simulink model "single_phase_ttype_inverter_param"  (R2026a)
settings: Solver=ode23tb  StopTime=param.sim.simlength  FixedStep=tc  MaxStep=param.glb_time.tc
values from neighbouring files (symbols this model uses):
  param = add_template_extras(param, options)    [init_model.m]
undefined symbols (not defined in the file or in its folder): delta_fht1, Ld_fht1, omega_fht1, ts_inv, Vac_FS, Vdc_nom, Xbez
libraries: fl_lib x36, nesl_utility x18, single_phase_transformer_lib x3, phase_shift_filter_ccaller x2, dclink_for_three_levels x1, three_phase_voltage_emulator x1, power_meter_iec x1, single_phase_transformer x1, three_phase_diode_rectifier x1, three_phase_diode_rectifier_with_thermal_model x1, full_bridge_three_level_ttype_ideal_switch_based_model x1, full_bridge_three_level_ttype_mosfet_based_model x1
(part 3 of 4)

== system single_phase_ttype_inverter_param/single_phase_inverter/single phase inverter control/single_phase_inverter_ctrl/phase generator/dq_pll_ccaller/first_harmonic_tracker1 ==
  u : Inport
  Bus Selector : BusSelector  OutputSignals=output_pu_hat
  Constant : Constant  Value=param.glb_time.ts_inv
  Constant1 : Constant  Value=0
  Constant2 : Constant  Value=param.afe.ctrl.fht_grid.omega_fht
  Constant3 : Constant  Value=param.afe.ctrl.fht_grid.delta_fht
  Constant4 : Constant  Value=param.afe.ctrl.fht_grid.Ld_fht(1)
  Constant5 : Constant  Value=param.afe.ctrl.fht_grid.Ld_fht(2)
  Data Type Conversion{1..2,6..9} (6 alike) : DataTypeConversion  OutDataTypeStr=single  SaturateOnIntegerOverflow=off  RndMeth=Floor
  Data Type Conversion3 : DataTypeConversion  OutDataTypeStr=uint8  SaturateOnIntegerOverflow=off  RndMeth=Floor
  Data Type Conversion4 : DataTypeConversion  OutDataTypeStr=double  SaturateOnIntegerOverflow=off  RndMeth=Floor
  Data Type Conversion5 : DataTypeConversion  OutDataTypeStr=uint8  SaturateOnIntegerOverflow=off  RndMeth=Floor
  Step : Step  Time=0.0125  InitialValue=1  FinalValue=0
  first_harmonic_tracker : CCaller  FunctionName=first_harmonic_tracker_process_simulink  PortSpecificationStruct="%)30     .    B \\   8    (     @         %    \"     D    !     0         %  0 \"0    $    _    07)G3F%M90  4&]R=$YA;64 4V-O<&4     26YD97@     5'EP90      4VEZ90      27-';&]B86P   X    P    !@    @    $          4    (     0    ,    !         !   P!O=70 #@   #     &    \"     0         !0    @    !     P    $         $  # &]U=  .    .     8    (    !          %    \"     $    &     0         0  ...(+4988 chars)"
  u_hat : Outport
  wires:
  Data Type Conversion4/1 -> u_hat/1
  Data Type Conversion3/1 -> first_harmonic_tracker/1
  Data Type Conversion1/1 -> first_harmonic_tracker/3
  Data Type Conversion2/1 -> first_harmonic_tracker/2
  first_harmonic_tracker/1 -> Bus Selector/1
  Bus Selector/1 -> Data Type Conversion4/1  "<output_pu_hat>"
  Step/1 -> Data Type Conversion3/1
  u/1 -> Data Type Conversion2/1
  Constant/1 -> Data Type Conversion1/1
  Constant1/1 -> Data Type Conversion5/1
  Data Type Conversion5/1 -> first_harmonic_tracker/8
  Constant2/1 -> Data Type Conversion6/1
  Data Type Conversion6/1 -> first_harmonic_tracker/4
  Constant3/1 -> Data Type Conversion7/1
  Data Type Conversion7/1 -> first_harmonic_tracker/5
  Constant4/1 -> Data Type Conversion8/1
  Data Type Conversion8/1 -> first_harmonic_tracker/6
  Constant5/1 -> Data Type Conversion9/1
  Data Type Conversion9/1 -> first_harmonic_tracker/7

== system single_phase_ttype_inverter_param/single_phase_inverter/single phase inverter control/single_phase_inverter_ctrl/phase generator/dq_pll_ccaller/first_harmonic_tracker2 ==
  u : Inport
  Bus Selector : BusSelector  OutputSignals=output_pu_hat
  Constant : Constant  Value=param.glb_time.ts_inv
  Constant1 : Constant  Value=2
  Constant2 : Constant  Value=param.afe.ctrl.fht_grid.omega_fht
  Constant3 : Constant  Value=param.afe.ctrl.fht_grid.delta_fht
  Constant4 : Constant  Value=param.afe.ctrl.fht_grid.Ld_fht(1)
  Constant5 : Constant  Value=param.afe.ctrl.fht_grid.Ld_fht(2)
  Data Type Conversion{1..2,6..9} (6 alike) : DataTypeConversion  OutDataTypeStr=single  SaturateOnIntegerOverflow=off  RndMeth=Floor
  Data Type Conversion3 : DataTypeConversion  OutDataTypeStr=uint8  SaturateOnIntegerOverflow=off  RndMeth=Floor
  Data Type Conversion4 : DataTypeConversion  OutDataTypeStr=double  SaturateOnIntegerOverflow=off  RndMeth=Floor
  Data Type Conversion5 : DataTypeConversion  OutDataTypeStr=uint8  SaturateOnIntegerOverflow=off  RndMeth=Floor
  Step : Step  Time=0.0125  InitialValue=1  FinalValue=0
  first_harmonic_tracker : CCaller  FunctionName=first_harmonic_tracker_process_simulink  PortSpecificationStruct="%)30     .    B \\   8    (     @         %    \"     D    !     0         %  0 \"0    $    _    07)G3F%M90  4&]R=$YA;64 4V-O<&4     26YD97@     5'EP90      4VEZ90      27-';&]B86P   X    P    !@    @    $          4    (     0    ,    !         !   P!O=70 #@   #     &    \"     0         !0    @    !     P    $         $  # &]U=  .    .     8    (    !          %    \"     $    &     0         0  ...(+4988 chars)"
  u_hat : Outport
  wires:
  Data Type Conversion9/1 -> first_harmonic_tracker/7
  Constant5/1 -> Data Type Conversion9/1
  Data Type Conversion8/1 -> first_harmonic_tracker/6
  Constant4/1 -> Data Type Conversion8/1
  Data Type Conversion7/1 -> first_harmonic_tracker/5
  Constant3/1 -> Data Type Conversion7/1
  Data Type Conversion6/1 -> first_harmonic_tracker/4
  Constant2/1 -> Data Type Conversion6/1
  Data Type Conversion5/1 -> first_harmonic_tracker/8
  Constant1/1 -> Data Type Conversion5/1
  Constant/1 -> Data Type Conversion1/1
  u/1 -> Data Type Conversion2/1
  Step/1 -> Data Type Conversion3/1
  Bus Selector/1 -> Data Type Conversion4/1  "<output_pu_hat>"
  first_harmonic_tracker/1 -> Bus Selector/1
  Data Type Conversion2/1 -> first_harmonic_tracker/2
  Data Type Conversion1/1 -> first_harmonic_tracker/3
  Data Type Conversion3/1 -> first_harmonic_tracker/1
  Data Type Conversion4/1 -> u_hat/1

== system single_phase_ttype_inverter_param/single_phase_inverter/single phase inverter control/single_phase_inverter_ctrl/phase generator/dq_pll_ccaller/first_harmonic_tracker3 ==
  u : Inport
  Bus Selector : BusSelector  OutputSignals=output_pu_hat
  Constant : Constant  Value=param.glb_time.ts_inv
  Constant1 : Constant  Value=4
  Constant2 : Constant  Value=param.afe.ctrl.fht_grid.omega_fht
  Constant3 : Constant  Value=param.afe.ctrl.fht_grid.delta_fht
  Constant4 : Constant  Value=param.afe.ctrl.fht_grid.Ld_fht(1)
  Constant5 : Constant  Value=param.afe.ctrl.fht_grid.Ld_fht(2)
  Data Type Conversion{1..2,6..9} (6 alike) : DataTypeConversion  OutDataTypeStr=single  SaturateOnIntegerOverflow=off  RndMeth=Floor
  Data Type Conversion3 : DataTypeConversion  OutDataTypeStr=uint8  SaturateOnIntegerOverflow=off  RndMeth=Floor
  Data Type Conversion4 : DataTypeConversion  OutDataTypeStr=double  SaturateOnIntegerOverflow=off  RndMeth=Floor
  Data Type Conversion5 : DataTypeConversion  OutDataTypeStr=uint8  SaturateOnIntegerOverflow=off  RndMeth=Floor
  Step : Step  Time=0.0125  InitialValue=1  FinalValue=0
  first_harmonic_tracker : CCaller  FunctionName=first_harmonic_tracker_process_simulink  PortSpecificationStruct="%)30     .    B \\   8    (     @         %    \"     D    !     0         %  0 \"0    $    _    07)G3F%M90  4&]R=$YA;64 4V-O<&4     26YD97@     5'EP90      4VEZ90      27-';&]B86P   X    P    !@    @    $          4    (     0    ,    !         !   P!O=70 #@   #     &    \"     0         !0    @    !     P    $         $  # &]U=  .    .     8    (    !          %    \"     $    &     0         0  ...(+4988 chars)"
  u_hat : Outport
  wires:
  Data Type Conversion4/1 -> u_hat/1
  Data Type Conversion3/1 -> first_harmonic_tracker/1
  Data Type Conversion1/1 -> first_harmonic_tracker/3
  Data Type Conversion2/1 -> first_harmonic_tracker/2
  first_harmonic_tracker/1 -> Bus Selector/1
  Bus Selector/1 -> Data Type Conversion4/1  "<output_pu_hat>"
  Step/1 -> Data Type Conversion3/1
  u/1 -> Data Type Conversion2/1
  Constant/1 -> Data Type Conversion1/1
  Constant1/1 -> Data Type Conversion5/1
  Data Type Conversion5/1 -> first_harmonic_tracker/8
  Constant2/1 -> Data Type Conversion6/1
  Data Type Conversion6/1 -> first_harmonic_tracker/4
  Constant3/1 -> Data Type Conversion7/1
  Data Type Conversion7/1 -> first_harmonic_tracker/5
  Constant4/1 -> Data Type Conversion8/1
  Data Type Conversion8/1 -> first_harmonic_tracker/6
  Constant5/1 -> Data Type Conversion9/1
  Data Type Conversion9/1 -> first_harmonic_tracker/7

== system single_phase_ttype_inverter_param/single_phase_inverter/single phase inverter control/single_phase_inverter_ctrl/single_phase_current_control/dqpi_current_controller/alphabeta2dq ==
  alpha : Inport
  beta : Inport  Port=2
  MATLAB Function : MATLAB Function  TreatAsAtomicUnit=on
  "d " : Outport  VectorParamsAs1DForOutWhenUnconnected=off
  "q " : Outport  Port=2  VectorParamsAs1DForOutWhenUnconnected=off
  wires:
  alpha/1 -> MATLAB Function/1(alpha)
  beta/1 -> MATLAB Function/2(beta)
  MATLAB Function/1(d) -> "d "/1
  MATLAB Function/2(q) -> "q "/1
  [phase] -> MATLAB Function/3(phase)

== system single_phase_ttype_inverter_param/single_phase_inverter/single phase inverter control/single_phase_inverter_ctrl/single_phase_current_control/dqpi_current_controller/dq2alphabeta ==
  d : Inport
  q : Inport  Port=2
  MATLAB Function : MATLAB Function  TreatAsAtomicUnit=on
  alpha : Outport  VectorParamsAs1DForOutWhenUnconnected=off
  wires:
  d/1 -> MATLAB Function/1(d)
  q/1 -> MATLAB Function/2(q)
  MATLAB Function/1(alpha) -> alpha/1
  [phase] -> MATLAB Function/3(phase)

== system single_phase_ttype_inverter_param/single_phase_inverter/single phase inverter control/single_phase_inverter_ctrl/single_phase_current_control/dqpi_current_controller/dq_vector_pi ==
  id_ref : Inport
  id : Inport  Port=2
  iq : Inport  Port=3
  iq_ref : Inport  Port=4
  dq_vector_pi : dq_vector_pi/dq_vector_pi  kp=param.spinv.ctrl.kp_inv  ki=param.spinv.ctrl.ki_inv  ts=param.glb_time.ts_inv  lim_ctrl_out=1  CTRPIFF_CLIP_RELEASE=1e-3
  ud_ctrl : Outport
  uq_ctrl : Outport  Port=2
  wires:
  id_ref/1 -> dq_vector_pi/1  "id_ref"
  iq_ref/1 -> dq_vector_pi/3  "iq_ref"
  dq_vector_pi/1 -> ud_ctrl/1  "ud_ctrl"
  iq/1 -> dq_vector_pi/4  "iq"
  id/1 -> dq_vector_pi/2  "id"
  dq_vector_pi/2 -> uq_ctrl/1  "uq_ctrl"
  [dclink_voltage_pu] -> dq_vector_pi/5

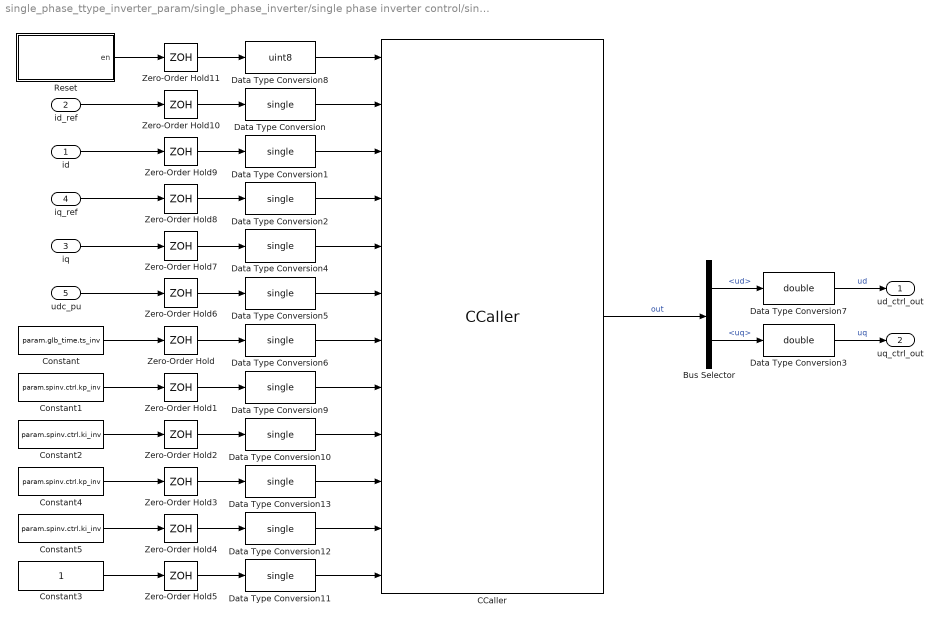
== system single_phase_ttype_inverter_param/single_phase_inverter/single phase inverter control/single_phase_inverter_ctrl/single_phase_current_control/dqpi_current_controller/dq_vector_pi_ccaller ==
  id : Inport
  id_ref : Inport  Port=2
  iq : Inport  Port=3
  iq_ref : Inport  Port=4
  udc_pu : Inport  Port=5
  Bus Selector : BusSelector  OutputSignals=ud,uq
  CCaller : CCaller  FunctionName=dqvector_pi_process_simulink  PortSpecificationStruct="%)30     .    ,!8   8    (     @         %    \"     T    !     0         %  0 \"0    $    _    07)G3F%M90  4&]R=$YA;64 4V-O<&4     26YD97@     5'EP90      4VEZ90      27-';&]B86P   X    P    !@    @    $          4    (     0    ,    !         !   P!O=70 #@   #     &    \"     0         !0    @    !     P    $         $  # &]U=  .    .     8    (    !          %    \"     $    &     0         0   ...(+7280 chars)"
  Constant : Constant  Value=param.glb_time.ts_inv
  Constant1 : Constant  Value=param.spinv.ctrl.kp_inv
  Constant2 : Constant  Value=param.spinv.ctrl.ki_inv
  Constant3 : Constant
  Constant4 : Constant  Value=param.spinv.ctrl.kp_inv
  Constant5 : Constant  Value=param.spinv.ctrl.ki_inv
  Data Type Conversion{,1..2,4..6,9..13} (11 alike) : DataTypeConversion  OutDataTypeStr=single  SaturateOnIntegerOverflow=off  RndMeth=Floor
  Data Type Conversion3 : DataTypeConversion  OutDataTypeStr=double  SaturateOnIntegerOverflow=off  RndMeth=Floor
  Data Type Conversion7 : DataTypeConversion  OutDataTypeStr=double  SaturateOnIntegerOverflow=off  RndMeth=Floor
  Data Type Conversion8 : DataTypeConversion  OutDataTypeStr=uint8  SaturateOnIntegerOverflow=off  RndMeth=Floor
  Reset : Subsystem
  Zero-Order Hold{,1..11} (12 alike) : ZeroOrderHold  SampleTime=-1
  ud_ctrl_out : Outport
  uq_ctrl_out : Outport  Port=2
  wires:
  Data Type Conversion5/1 -> CCaller/6
  Data Type Conversion/1 -> CCaller/2
  CCaller/1 -> Bus Selector/1  "out"
  Data Type Conversion1/1 -> CCaller/3
  Data Type Conversion4/1 -> CCaller/5
  Data Type Conversion2/1 -> CCaller/4
  Data Type Conversion6/1 -> CCaller/7
  Bus Selector/2 -> Data Type Conversion3/1  "<uq>"
  Bus Selector/1 -> Data Type Conversion7/1  "<ud>"
  Data Type Conversion7/1 -> ud_ctrl_out/1  "ud"
  Data Type Conversion3/1 -> uq_ctrl_out/1  "uq"
  Data Type Conversion8/1 -> CCaller/1
  Data Type Conversion9/1 -> CCaller/8
  Data Type Conversion10/1 -> CCaller/9
  Data Type Conversion11/1 -> CCaller/12
  Data Type Conversion13/1 -> CCaller/10
  Data Type Conversion12/1 -> CCaller/11
  Constant3/1 -> Zero-Order Hold5/1
  Constant5/1 -> Zero-Order Hold4/1
  Constant4/1 -> Zero-Order Hold3/1
  Constant2/1 -> Zero-Order Hold2/1
  Constant1/1 -> Zero-Order Hold1/1
  Constant/1 -> Zero-Order Hold/1
  udc_pu/1 -> Zero-Order Hold6/1
  iq/1 -> Zero-Order Hold7/1
  iq_ref/1 -> Zero-Order Hold8/1
  Reset/1(en) -> Zero-Order Hold11/1
  id_ref/1 -> Zero-Order Hold10/1
  id/1 -> Zero-Order Hold9/1
  Zero-Order Hold/1 -> Data Type Conversion6/1
  Zero-Order Hold1/1 -> Data Type Conversion9/1
  Zero-Order Hold2/1 -> Data Type Conversion10/1
  Zero-Order Hold3/1 -> Data Type Conversion13/1
  Zero-Order Hold4/1 -> Data Type Conversion12/1
  Zero-Order Hold5/1 -> Data Type Conversion11/1
  Zero-Order Hold6/1 -> Data Type Conversion5/1
  Zero-Order Hold7/1 -> Data Type Conversion4/1
  Zero-Order Hold8/1 -> Data Type Conversion2/1
  Zero-Order Hold9/1 -> Data Type Conversion1/1
  Zero-Order Hold10/1 -> Data Type Conversion/1
  Zero-Order Hold11/1 -> Data Type Conversion8/1

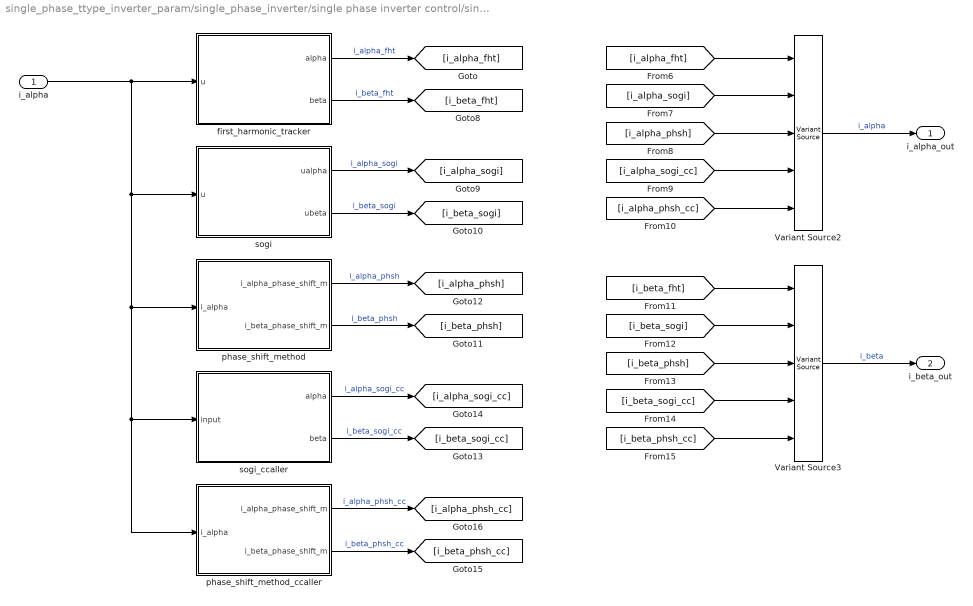
== system single_phase_ttype_inverter_param/single_phase_inverter/single phase inverter control/single_phase_inverter_ctrl/single_phase_current_control/dqpi_current_controller/i2alphabeta ==
  i_alpha : Inport
  Variant Source2 : VariantSource  VariantControls="{param.spinv.impl.use_single_phase_inverter_based_FHT == 1, param.spinv.impl.use_single_phase_inverter_based_SOGI  == 1, param.spinv.impl.use_single_phase_inverter_based_PHSH  == 1, param.spinv.impl.use_single_phase_inverter_based_SOGI_ccaller  == 1, param.spinv.impl.use_single_phase_inverter_based_PHSH_ccaller  == 1}"
  Variant Source3 : VariantSource  VariantControls="{param.spinv.impl.use_single_phase_inverter_based_FHT == 1, param.spinv.impl.use_single_phase_inverter_based_SOGI  == 1, param.spinv.impl.use_single_phase_inverter_based_PHSH  == 1, param.spinv.impl.use_single_phase_inverter_based_SOGI_ccaller  == 1, param.spinv.impl.use_single_phase_inverter_based_PHSH_ccaller  == 1}"
  first_harmonic_tracker : Subsystem
  phase_shift_method : Subsystem
  phase_shift_method_ccaller : Subsystem
  sogi : Subsystem
  sogi_ccaller : Subsystem
  i_alpha_out : Outport
  i_beta_out : Outport  Port=2
  wires:
  i_alpha/1 -> phase_shift_method_ccaller/1(i_alpha), sogi_ccaller/1(input), phase_shift_method/1(i_alpha), sogi/1(u), first_harmonic_tracker/1(u)
  [i_alpha_phsh] -> Variant Source2/3
  [i_beta_sogi] -> Variant Source3/2
  [i_alpha_phsh_cc] -> Variant Source2/5
  first_harmonic_tracker/2(beta) -> [i_beta_fht]  "i_beta_fht"
  phase_shift_method/2(i_beta_phase_shift_m) -> [i_beta_phsh]  "i_beta_phsh"
  phase_shift_method/1(i_alpha_phase_shift_m) -> [i_alpha_phsh]  "i_alpha_phsh"
  [i_alpha_sogi] -> Variant Source2/2
  phase_shift_method_ccaller/1(i_alpha_phase_shift_m) -> [i_alpha_phsh_cc]  "i_alpha_phsh_cc"
  [i_beta_phsh_cc] -> Variant Source3/5
  [i_alpha_fht] -> Variant Source2/1
  [i_beta_phsh] -> Variant Source3/3
  sogi_ccaller/1(alpha) -> [i_alpha_sogi_cc]  "i_alpha_sogi_cc"
  [i_beta_sogi_cc] -> Variant Source3/4
  sogi/1(ualpha) -> [i_alpha_sogi]  "i_alpha_sogi"
  sogi/2(ubeta) -> [i_beta_sogi]  "i_beta_sogi"
  phase_shift_method_ccaller/2(i_beta_phase_shift_m) -> [i_beta_phsh_cc]  "i_beta_phsh_cc"
  sogi_ccaller/2(beta) -> [i_beta_sogi_cc]  "i_beta_sogi_cc"
  Variant Source2/1 -> i_alpha_out/1  "i_alpha"
  first_harmonic_tracker/1(alpha) -> [i_alpha_fht]  "i_alpha_fht"
  [i_alpha_sogi_cc] -> Variant Source2/4
  [i_beta_fht] -> Variant Source3/1
  Variant Source3/1 -> i_beta_out/1  "i_beta"

== system single_phase_ttype_inverter_param/single_phase_inverter/single phase inverter control/single_phase_inverter_ctrl/single_phase_current_control/rpi_current_controller/Reset ==
  Step : Step  Time=0.05  InitialValue=1  FinalValue=0
  en : Outport
  wires:
  Step/1 -> en/1

== system single_phase_ttype_inverter_param/single_phase_inverter/single phase inverter control/single_phase_inverter_ctrl/sistem_identification/open loop u//f/dq2alphabeta ==
  Constant1 : Constant  Value=0
  Data Store Read : DataStoreRead  DataStoreName=u_test  IndexOptions=Index vector (dialog)  Indices=1  OutputSizes=1
  MATLAB Function : MATLAB Function  TreatAsAtomicUnit=on
  alpha : Outport  VectorParamsAs1DForOutWhenUnconnected=off
  wires:
  [phase] -> MATLAB Function/3(phase)
  MATLAB Function/1(alpha) -> alpha/1
  Data Store Read/1 -> MATLAB Function/1(d)
  Constant1/1 -> MATLAB Function/2(q)

== system single_phase_ttype_inverter_param/single_phase_inverter/single phase inverter control/single_phase_inverter_ctrl/sistem_identification/open loop u//f/first_harmonic_tracker ==
  u : Inport
  Bus Selector : BusSelector  OutputSignals=output_pu_hat,output_pu_hat_dot
  Constant : Constant  Value=ts_inv
  Constant1 : Constant  Value=8
  Constant2 : Constant  Value=omega_fht1
  Constant3 : Constant  Value=delta_fht1
  Constant4 : Constant  Value=Ld_fht1(1)
  Constant5 : Constant  Value=Ld_fht1(2)
  Data Type Conversion{1..2,6..9} (6 alike) : DataTypeConversion  OutDataTypeStr=single  SaturateOnIntegerOverflow=off  RndMeth=Floor
  Data Type Conversion10 : DataTypeConversion  OutDataTypeStr=double  SaturateOnIntegerOverflow=off  RndMeth=Floor
  Data Type Conversion3 : DataTypeConversion  OutDataTypeStr=uint8  SaturateOnIntegerOverflow=off  RndMeth=Floor
  Data Type Conversion4 : DataTypeConversion  OutDataTypeStr=double  SaturateOnIntegerOverflow=off  RndMeth=Floor
  Data Type Conversion5 : DataTypeConversion  OutDataTypeStr=uint8  SaturateOnIntegerOverflow=off  RndMeth=Floor
  Gain : Gain  Gain=-1/omega_fht1
  Step : Step  Time=0.0125  InitialValue=1  FinalValue=0
  first_harmonic_tracker : CCaller  FunctionName=first_harmonic_tracker_process_simulink  PortSpecificationStruct="%)30     .    B \\   8    (     @         %    \"     D    !     0         %  0 \"0    $    _    07)G3F%M90  4&]R=$YA;64 4V-O<&4     26YD97@     5'EP90      4VEZ90      27-';&]B86P   X    P    !@    @    $          4    (     0    ,    !         !   P!O=70 #@   #     &    \"     0         !0    @    !     P    $         $  # &]U=  .    .     8    (    !          %    \"     $    &     0         0  ...(+4988 chars)"
  alpha : Outport
  beta : Outport  Port=2
  wires:
  Data Type Conversion4/1 -> alpha/1
  Data Type Conversion3/1 -> first_harmonic_tracker/1
  Data Type Conversion1/1 -> first_harmonic_tracker/3
  Data Type Conversion2/1 -> first_harmonic_tracker/2
  first_harmonic_tracker/1 -> Bus Selector/1
  Bus Selector/1 -> Data Type Conversion4/1  "<output_pu_hat>"
  Step/1 -> Data Type Conversion3/1
  u/1 -> Data Type Conversion2/1
  Constant/1 -> Data Type Conversion1/1
  Constant1/1 -> Data Type Conversion5/1
  Data Type Conversion5/1 -> first_harmonic_tracker/8
  Constant2/1 -> Data Type Conversion6/1
  Data Type Conversion6/1 -> first_harmonic_tracker/4
  Constant3/1 -> Data Type Conversion7/1
  Data Type Conversion7/1 -> first_harmonic_tracker/5
  Constant4/1 -> Data Type Conversion8/1
  Data Type Conversion8/1 -> first_harmonic_tracker/6
  Constant5/1 -> Data Type Conversion9/1
  Data Type Conversion9/1 -> first_harmonic_tracker/7
  Bus Selector/2 -> Data Type Conversion10/1  "<output_pu_hat_dot>"
  Data Type Conversion10/1 -> Gain/1
  Gain/1 -> beta/1

== system single_phase_ttype_inverter_param/single_phase_inverter/single phase inverter control/single_phase_inverter_ctrl/sistem_identification/open loop u//f/module ==
  i_alpha : Inport
  i_beta : Inport  Port=2
  Sqrt : Sqrt
  Square : Math  Operator=square
  Square1 : Math  Operator=square
  Sum : Sum  Inputs=|++
  i : Outport
  wires:
  i_beta/1 -> Square1/1
  i_alpha/1 -> Square/1
  Square/1 -> Sum/1
  Sum/1 -> Sqrt/1
  Square1/1 -> Sum/2
  Sqrt/1 -> i/1  "i"
